simulink library "multicopter_aerodynamics_simple_lib"  (R2018b)
settings: Solver=VariableStepAuto  StartTime=0.0  StopTime=10.0  RelTol=1e-3
undefined symbols (not defined in the file): copter, copterAero
libraries: flight_parameters_lib x4, aerodynamics_lib x1, axes_transformation_lib x1
settings Model: Creator=Ybeyer  LastModifiedBy=yannic
settings SFSimCC: SimUseLocalCustomCode=off
settings RTWCC: RTWUseLocalCustomCode=off
settings CodeAppCC: StateflowObjectComments=on

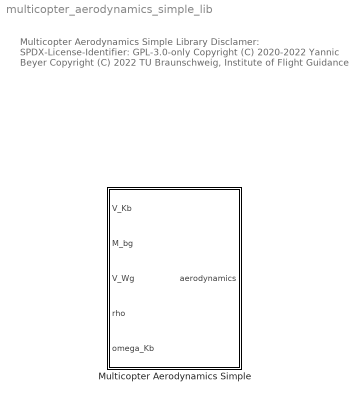
== system multicopter_aerodynamics_simple_lib ==
  note: Multicopter Aerodynamics Simple Library
      |
      | Disclamer:
      | SPDX-License-Identifier: GPL-3.0-only
      |
      | Copyright (C) 2020-2022 Yannic Beyer
      | Copyright (C) 2022 TU Braunschweig, Institute of Flight Guidance
  Multicopter Aerodynamics Simple : Subsystem  mask{copterAero=copterAero}
      mask prompts: copterAero "aerodynamics parameters struct"
      mask DialogControl DescGroupVar Prompt: Multicopter Aerodynamics Simple
      mask DialogControl DescTextVar Prompt: The simple multicopter aerodynamics model is described in:
      mask DialogControl Control2 Prompt: Beyer, Y. (2016): Flugmechanische Modellierung von Multicopter-Systemen in MATLAB/Simulink, Studienarbeit, TU Braunschweig, Institut für Flugführung.

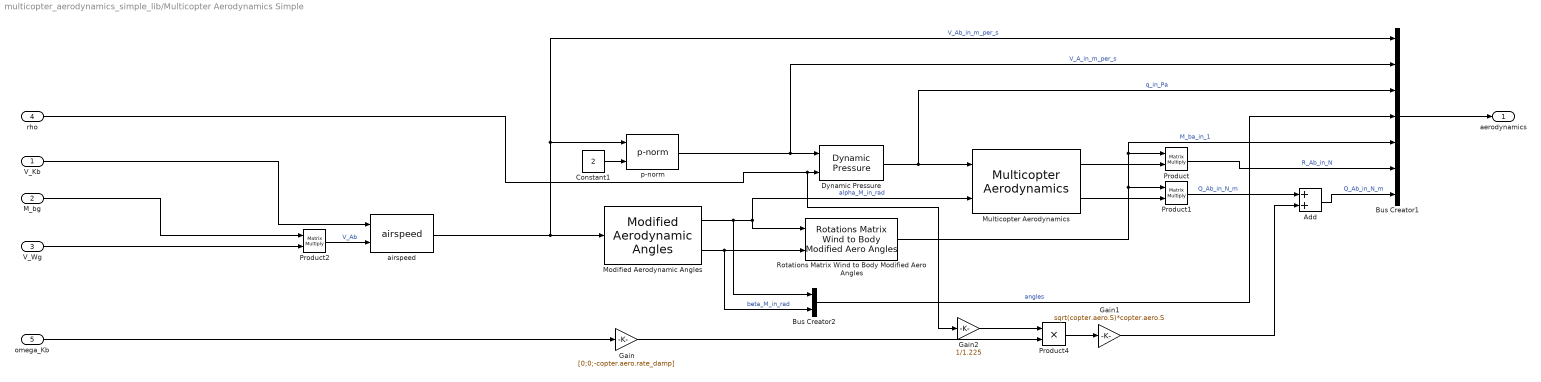
== system multicopter_aerodynamics_simple_lib/Multicopter Aerodynamics Simple ==
  V_Kb : Inport
  M_bg : Inport  Port=2
  V_Wg : Inport  Port=3  OutDataTypeStr=double  PortDimensions=3
  rho : Inport  Port=4  OutDataTypeStr=double  PortDimensions=1
  omega_Kb : Inport  Port=5  OutDataTypeStr=double  PortDimensions=3
  Add : Sum
  Bus Creator1 : BusCreator  Inputs=7
  Bus Creator2 : BusCreator  Inputs=2
  Constant1 : Constant  Value=2
  Dynamic Pressure : flight_parameters_lib/Dynamic Pressure
      settings: SourceProductName=LADAC
  Gain : Gain  Gain=[0;0;-copter.aero.rate_damp]
  Gain1 : Gain  Gain=sqrt(copter.aero.S)*copter.aero.S
  Gain2 : Gain  Gain=1/1.225
  Modified Aerodynamic Angles : flight_parameters_lib/Modified Aerodynamic Angles  SystemSampleTime=-1
      settings: SourceProductName=LADAC
  Multicopter Aerodynamics : aerodynamics_lib/Multicopter Aerodynamics  S=copterAero.S  C_D_max=copterAero.C_Dmax  C_D_min=copterAero.C_Dmin  C_L_max=copterAero.C_Lmax  x_CoP_b=copterAero.CoP_xy  z_CoP_b=copterAero.CoP_z
      settings: SourceProductName=LADAC
  Product : Product  Multiplication=Matrix(*)
  Product1 : Product  Multiplication=Matrix(*)
  Product2 : Product  Multiplication=Matrix(*)
  Product4 : Product
  Rotations Matrix Wind to Body Modified Aero Angles : axes_transformation_lib/Rotations Matrix Wind to Body Modified Aero Angles  SystemSampleTime=-1
      settings: SourceProductName=LADAC
  airspeed : flight_parameters_lib/airspeed
      settings: SourceProductName=LADAC
  p-norm : flight_parameters_lib/p-norm  SystemSampleTime=-1
      settings: SourceProductName=LADAC
  aerodynamics : Outport
  wires:
  Product/1 -> Bus Creator1/6  "R_Ab_in_N"
  rho/1 -> Gain2/1, Dynamic Pressure/2
  Add/1 -> Bus Creator1/7  "Q_Ab_in_N_m"
  V_Wg/1 -> Product2/2
  Dynamic Pressure/1 -> Multicopter Aerodynamics/1, Bus Creator1/3  "q_in_Pa"
  Multicopter Aerodynamics/1 -> Product/2
  Modified Aerodynamic Angles/2 -> Rotations Matrix Wind to Body Modified Aero Angles/2, Bus Creator2/2  "beta_M_in_rad"
  Rotations Matrix Wind to Body Modified Aero Angles/1 -> Product/1, Bus Creator1/5, Product1/1  "M_ba_in_1"
  airspeed/1 -> Modified Aerodynamic Angles/1, p-norm/1, Bus Creator1/1  "V_Ab_in_m_per_s"
  Modified Aerodynamic Angles/1 -> Multicopter Aerodynamics/2, Rotations Matrix Wind to Body Modified Aero Angles/1, Bus Creator2/1  "alpha_M_in_rad"
  Bus Creator2/1 -> Bus Creator1/4  "angles"
  p-norm/1 -> Dynamic Pressure/1, Bus Creator1/2  "V_A_in_m_per_s"
  M_bg/1 -> Product2/1
  Product2/1 -> airspeed/2  "V_Ab"
  V_Kb/1 -> airspeed/1
  Constant1/1 -> p-norm/2
  Bus Creator1/1 -> aerodynamics/1
  Multicopter Aerodynamics/2 -> Product1/2
  Product1/1 -> Add/1  "Q_Ab_in_N_m"
  Product4/1 -> Gain1/1
  omega_Kb/1 -> Gain/1
  Gain/1 -> Product4/2
  Gain1/1 -> Add/2
  Gain2/1 -> Product4/1
